simulink model "DWPT_simscape"  (R2026b)
settings: Solver=ode23t  StopTime=0.07  FixedStep=Ts  MaxStep=1.0E-7
InitFcn:
  | f = 85000;
  | Fs = 100000000;       % 100
  | Ts = 1/Fs;          % 步长
  | 
  | 
  | fprintf('周期/Ts = %.10f (应=100)\n', (1/f)/Ts);
  | 
  | 
  | LP1 = 437.3e-6;
  | LP2 = 420.6e-6;
  | LS = 306e-6;
  | LT1 = 98e-6;
  | LT2 = 99.5e-6;
  | 
  | CP1 = 9.03e-9;
  | CP2 = 9.23e-9;
  | 
  | CT1 = 55e-9;
  | CT2 = 54e-9;
  | CS = 12.5e-9;
  | 
  | M1  = 94e-6;
  | M2  = 0e-6;
  | 
  | RP1 = 1.4;
  | RP2 = 1.4;
  | RS = 1.3;
  | 
  | RL = 30;
undefined symbols (not defined in the file): Lf, Lt, M, Mosfet_class, MutualInductance_class, UniversalBridge_class
libraries: fl_lib x30, nesl_utility x23, ee_lib x9, eeRmsMeasurement x7, eeGeneralControl x3, dspfdesign x1, elec_conv_HighZElecRef x1, spspowerguiLib x1
(part 1 of 2)
settings Model: Creator=yihao  LastModifiedBy=rithvik
settings DataIOCC: ReturnWorkspaceOutputs=off
settings DebuggingCC: SaveWithParameterizedLinksMsg=none
settings RTWCC: GPUComputeCapability=5.0
settings SimscapeCC: SimscapeNominalValues="[{\"value\":\"1\",\"unit\":\"A\"},{\"value\":\"1\",\"unit\":\"bar\"},{\"value\":\"1\",\"unit\":\"cm^2\"},{\"value\":\"1\",\"unit\":\"cm^3/s\"},{\"value\":\"1\",\"unit\":\"kJ/kg\"},{\"value\":\"1\",\"unit\":\"kW\"},{\"value\":\"1\",\"unit\":\"l\"},{\"value\":\"1\",\"unit\":\"N\"},{\"value\":\"1\",\"unit\":\"N*m\"},{\"value\":\"1\",\"unit\":\"V\"},{\"value\":\"0.001\",\"unit\":\"Wb\"}]"  SimscapeUseEnergyAccounting=off

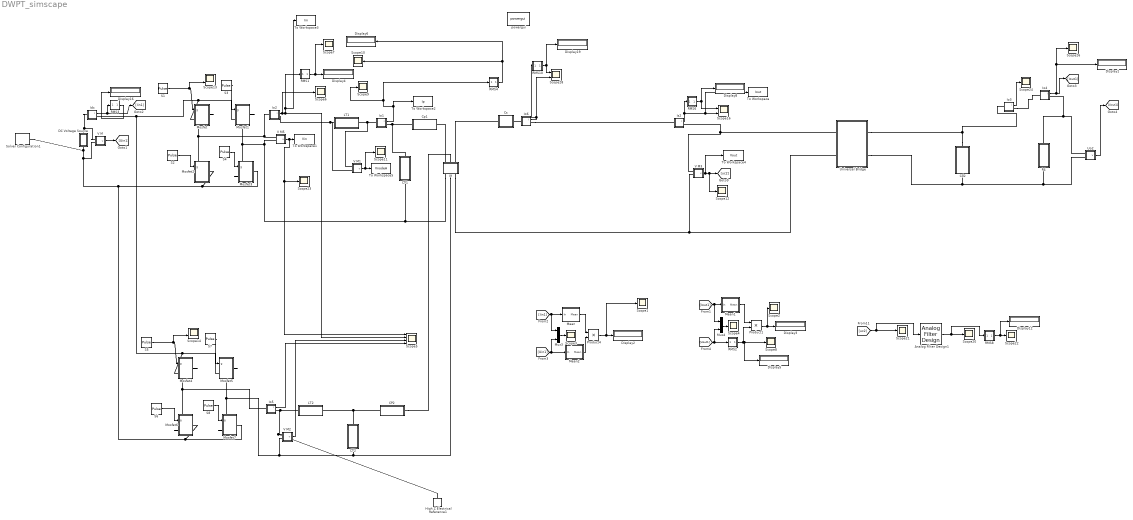
== system DWPT_simscape ==
  Analog Filter Design1 : dspfdesign/Analog Filter Design  method=Butterworth  filttype=Lowpass  N=8  Wlo=85000*2*pi  Whi=80  Rp=2  Rs=40
  CP2 : Subsystem
      settings: OpenFcn=elec.conv.unmask(gcb);
  CT1 : Subsystem
      settings: OpenFcn=elec.conv.unmask(gcb);
  CT2 : Subsystem
      settings: OpenFcn=elec.conv.unmask(gcb);
  Cd2 : Subsystem
      settings: OpenFcn=elec.conv.unmask(gcb);
  Cp1 : Subsystem
      settings: OpenFcn=elec.conv.unmask(gcb);
  Cs : Subsystem
      settings: OpenFcn=elec.conv.unmask(gcb);
  DC Voltage Source : Subsystem
      settings: OpenFcn=elec.conv.unmask(gcb);
  Display{1..6,8,12,16,19} (10 alike) : Display
  High Z Electrical Reference1 : elec_conv_HighZElecRef/High Z Electrical Reference  SystemSampleTime=-1  VariantActivationTime=update diagram  EmptyChoice=off  PassThrough=off  PassThroughVariantControl=(default)  EmptyChoiceVariantControl=(default)  AllowFlexibleInterface=on  Latency=0  AutoFrameSizeCalculation=off
  Idc : Subsystem
      settings: OpenFcn=elec.conv.unmask(gcb);
  Io1 : Subsystem
      settings: OpenFcn=elec.conv.unmask(gcb);
  Io2 : Subsystem
      settings: OpenFcn=elec.conv.unmask(gcb);
  Io3 : Subsystem
      settings: OpenFcn=elec.conv.unmask(gcb);
  Io4 : Subsystem
      settings: OpenFcn=elec.conv.unmask(gcb);
  Io5 : Subsystem
      settings: OpenFcn=elec.conv.unmask(gcb);
  Io6 : Subsystem
      settings: OpenFcn=elec.conv.unmask(gcb);
  Is2 : Subsystem
      settings: OpenFcn=elec.conv.unmask(gcb);
  LT1 : Subsystem
      settings: OpenFcn=elec.conv.unmask(gcb);
  LT2 : Subsystem
      settings: OpenFcn=elec.conv.unmask(gcb);
  M : Subsystem
      settings: AttributesFormatString=\n  OpenFcn=elec.conv.unmask(gcb);
  Mean : Subsystem
      settings: OpenFcn=elec.conv.unmask(gcb);
  Mean1 : Subsystem
      settings: OpenFcn=elec.conv.unmask(gcb);
  Mean2 : Subsystem
      settings: OpenFcn=elec.conv.unmask(gcb);
  Mosfet : Subsystem
      settings: OpenFcn=elec.conv.unmask(gcb);
  Mosfet1 : Subsystem
      settings: OpenFcn=elec.conv.unmask(gcb);
  Mosfet2 : Subsystem
      settings: OpenFcn=elec.conv.unmask(gcb);
  Mosfet3 : Subsystem
      settings: OpenFcn=elec.conv.unmask(gcb);
  Mosfet4 : Subsystem
      settings: OpenFcn=elec.conv.unmask(gcb);
  Mosfet5 : Subsystem
      settings: OpenFcn=elec.conv.unmask(gcb);
  Mosfet6 : Subsystem
      settings: OpenFcn=elec.conv.unmask(gcb);
  Mosfet7 : Subsystem
      settings: OpenFcn=elec.conv.unmask(gcb);
  Mux3 : Mux  Inputs=2
  Mux4 : Mux  Inputs=2
  Product1 : Product
  Product4 : Product
  R4 : Subsystem
      settings: OpenFcn=elec.conv.unmask(gcb);
  RMS1 : Subsystem
      settings: OpenFcn=elec.conv.unmask(gcb);
  RMS10 : Subsystem
      settings: OpenFcn=elec.conv.unmask(gcb);
  RMS2 : Subsystem
      settings: OpenFcn=elec.conv.unmask(gcb);
  RMS3 : Subsystem
      settings: OpenFcn=elec.conv.unmask(gcb);
  RMS4 : Subsystem
      settings: OpenFcn=elec.conv.unmask(gcb);
  RMS6 : Subsystem
      settings: OpenFcn=elec.conv.unmask(gcb);
  RMS8 : Subsystem
      settings: OpenFcn=elec.conv.unmask(gcb);
  S{1,4..5,8} (4 alike) : DiscretePulseGenerator  PulseType=Time based  Period=1/f  PulseWidth=49.5
  S{2..3,6..7} (4 alike) : DiscretePulseGenerator  PulseType=Time based  Period=1/f  PulseWidth=49.5  PhaseDelay=1/2/f
  Scope{1..4,6..12,20..24,26} (17 alike) : Scope
      Scope1 settings: ActiveDisplayYMinimum=-49.10464  ActiveDisplayYMaximum=441.94179  DataLoggingSaveFormat=Array
      Scope10 settings: ActiveDisplayYMinimum=-0.71464  ActiveDisplayYMaximum=6.43176  DataLoggingVariableName=ScopeData2  DataLoggingSaveFormat=Array
      Scope11 settings: ActiveDisplayYMinimum=-10.18584  ActiveDisplayYMaximum=11.18954  DataLoggingSaveFormat=Array
      Scope12 settings: ActiveDisplayYMinimum=-124.85082  ActiveDisplayYMaximum=124.97825  DataLoggingVariableName=ScopeData4  DataLoggingSaveFormat=Array
      Scope2 settings: ActiveDisplayYMinimum=-3.3359920538155139  ActiveDisplayYMaximum=30.023928484339635  DataLoggingVariableName=ScopeData12  DataLoggingSaveFormat=Array
      Scope20 settings: ActiveDisplayYMinimum=-998.97593  ActiveDisplayYMaximum=1003.83836  DataLoggingVariableName=ScopeData13  DataLoggingSaveFormat=Array
      Scope21 settings: ActiveDisplayYMinimum=-1098.42082  ActiveDisplayYMaximum=1097.9597  DataLoggingVariableName=ScopeData14  DataLoggingSaveFormat=Array
      Scope22 settings: ActiveDisplayYMinimum=-0.08617  ActiveDisplayYMaximum=0.77556  DataLoggingVariableName=ScopeData15  DataLoggingSaveFormat=Array
      Scope23 settings: ActiveDisplayYMinimum=-126.90541  ActiveDisplayYMaximum=126.90651  DataLoggingVariableName=ScopeData16  DataLoggingSaveFormat=Array
      Scope24 settings: ActiveDisplayYMinimum=-0.06956  ActiveDisplayYMaximum=0.62607  DataLoggingSaveFormat=Array
      Scope26 settings: ActiveDisplayYMinimum=-0.31456  ActiveDisplayYMaximum=2.83101  DataLoggingVariableName=ScopeData2  DataLoggingSaveFormat=Array
      Scope3 settings: ActiveDisplayYMinimum=-3742.24205  ActiveDisplayYMaximum=32139.40337  DataLoggingVariableName=ScopeData23  DataLoggingSaveFormat=Array
      Scope4 settings: ActiveDisplayYMinimum=-3.3830504056400548  ActiveDisplayYMaximum=30.4474536507605  DataLoggingVariableName=ScopeData27  DataLoggingSaveFormat=Array
      Scope6 settings: ActiveDisplayYMinimum=-10.18584  ActiveDisplayYMaximum=11.18954  DataLoggingVariableName=ScopeData29  DataLoggingSaveFormat=Array
      Scope7 settings: ActiveDisplayYMinimum=41.35748  ActiveDisplayYMaximum=44.91904  DataLoggingVariableName=ScopeData30  DataLoggingSaveFormat=Array
      Scope8 settings: ActiveDisplayYMinimum=-10.89533  ActiveDisplayYMaximum=134.54393  DataLoggingVariableName=ScopeData31  DataLoggingSaveFormat=Array
      Scope9 settings: ActiveDisplayYMinimum=-11.00674  ActiveDisplayYMaximum=11.77758  DataLoggingSaveFormat=Array
  Scope{13..14,16,28} (4 alike) : Scope  NumInputPorts=2
      Scope13 settings: ActiveDisplayYMinimum=-12.75848  ActiveDisplayYMaximum=112.74941  DataLoggingVariableName=ScopeData5  DataLoggingSaveFormat=Array
      Scope14 settings: ActiveDisplayYMinimum=-12.75848  ActiveDisplayYMaximum=112.74941  DataLoggingVariableName=ScopeData3  DataLoggingSaveFormat=Array
      Scope16 settings: ActiveDisplayYMinimum=-5.8521517419594016  ActiveDisplayYMaximum=5.8917781570828591  DataLoggingVariableName=ScopeData8  DataLoggingSaveFormat=Array
      Scope28 settings: ActiveDisplayYMinimum=-4.84326  ActiveDisplayYMaximum=4.41106  DataLoggingVariableName=ScopeData21  DataLoggingSaveFormat=Array
  Scope5 : Scope  NumInputPorts=4
      settings: ActiveDisplayYMinimum=-71.017946366553787  ActiveDisplayYMaximum=71.042097514829976  DataLoggingVariableName=ScopeData28  DataLoggingSaveFormat=Array
  Solver Configuration1 : nesl_utility/Solver Configuration  PhysicalDomain=network_engine_domain  SubClassName=solver  LeftPortType=input  RightPortType=generic  Tones=[]  Harmonics=[]  SimulateNoise=off  Profile=off  UseLocalSampling=off  EnableSwitchedLinearOptims=on  FrequencyDomain=off  UseCCode=off  RelTol=0.001  AbsTol=0.001  MinStep=1e-09  ToWorkspace=off  RevertToSquareIcSolve=off  NumHomotopyIterations=100  PhasorMode=off  PhasorModeNumHarmonics=1  ConsistencySolver=NEWTON_XTOL_AFTER_FTOL  CanonicalOrdering=CANONICAL  OptimizeIntermediates=OPTIMIZED  MulticoreSolverChoice=BACKWARD_EULER  IndexReductionMethod=DerivativeReplacement  DoDC=off  ResidualTolerance=1e-09  ConsistencyTolSource=GLOBAL  ConsistencyAbsTol=0.001  ConsistencyRelTol=0.001  ConsistencyTolFactor=0.001  UseLocalSolver=off  LocalSolverChoice=NE_BACKWARD_EULER_ADVANCER  ResolveIndetEquations=on  FunctionEvalNumThread=1  LocalSolverSampleTime=0.001  DoFixedCost=off  MaxNonlinIter=3  MaxModeIter=2  ComputeImpulses=off  ImpulseIterations=2  LinearAlgebra=auto  LinearAlgebraNumThread=0  EquationFormulation=NE_TIME_EF  DelaysMemoryBudget=1024  AutomaticFiltering=on  FilteringTimeConstant=0.001  PartitionStorageMethod=AS_NEEDED  PartitionMemoryBudget=1024  PartitionMethod=BALANCED  MultibodyUseLocalSolver=off  MultibodyLocalSolverChoice=ODE1  MultibodyLocalSolverSampleTime=0.001
  To Workspace : ToWorkspace  VariableName=Iout  SaveFormat=Structure With Time  SampleTime=-1
  To Workspace1 : ToWorkspace  VariableName=Vin  SaveFormat=Structure With Time  SampleTime=-1
  To Workspace2 : ToWorkspace  VariableName=Ip  SaveFormat=Structure With Time  SampleTime=-1
  To Workspace3 : ToWorkspace  VariableName=Iin  SaveFormat=Structure With Time  SampleTime=-1
  To Workspace4 : ToWorkspace  VariableName=Vout  SaveFormat=Structure With Time  SampleTime=-1
  To Workspace5 : ToWorkspace  VariableName=VnodeA  SaveFormat=Structure With Time  SampleTime=-1
  Universal Bridge : Subsystem
      settings: OpenFcn=elec.conv.unmask(gcb);
  Uo2 : Subsystem
      settings: OpenFcn=elec.conv.unmask(gcb);
  V M : Subsystem
      settings: OpenFcn=elec.conv.unmask(gcb);
  V M1 : Subsystem
      settings: OpenFcn=elec.conv.unmask(gcb);
  V M2 : Subsystem
      settings: OpenFcn=elec.conv.unmask(gcb);
  V M3 : Subsystem
      settings: OpenFcn=elec.conv.unmask(gcb);
  V M5 : Subsystem
      settings: OpenFcn=elec.conv.unmask(gcb);
  powergui : spspowerguiLib/powergui  Priority=1  SimulationMode=Discrete  SampleTime=1e-7  frequency=60  Iterations=50  frequencyindice=0  Pbase=100e6  ErrMax=1e-4  UnitsV=kV  UnitsW=MW  buscounter=0  FunctionMessages=off  echomessages=off  EnableUseOfTLC=off  CurrentSourceSwitches=off  DisableSnubberDevices=off  DisableRonSwitches=off  DisableVfSwitches=off  DisplayEquations=off  AutomaticDiscreteSolvers=off  SolverType=Tustin/Backward Euler (TBE)  Interpol=off  ExternalGateDelay=off  methode=off  Ts=100  x0status=blocks  SPID=on  SwTol=0  HookPort=off  NonlinearTolerance=1e-4  nMaxIteration=100  ContinueOnMaxIteration=off  RestoreLinks=warning  ResistiveCurrentMeasurement=off  Frange=[0:2:500]  Ylog=off  Xlog=on  ShowGrid=off  save=off  variable=ZData  structure=Is2  ZoomFFT=off  StartTime=0.1  cycles=5  DisplayStyle=1  fundamental=85000  FreqAxis=off  MaxFrequency=100000  frequencyindicesteady=1  RmsSteady=1  display=off
  wires:
  Is2/1(i) -> To Workspace/1, Scope16/2, RMS6/1(In)
  Io6/1(i) -> Scope28/2, RMS10/1(In)
  [Uin1] -> Mean2/1(In), Mux3/2
  V M5/1(v) -> To Workspace1/1, Scope5/1, Scope23/1
  [Uout1] -> RMS2/1(In), Mux4/2
  RMS4/1(RMS) -> Display6/1, Scope10/1
  Mean/1(Mean) -> Product4/1
  Idc/1(i) -> RMS3/1(In), [Iin1]
  V M3/1(v) -> To Workspace4/1, Scope12/1, [uc2]
  Mean1/1(Mean) -> Product1/1
  Io2/1(i) -> Scope5/2, To Workspace3/1, RMS1/1(In), Scope6/1
  [Iin1] -> Mean/1(In), Mux3/1
  S2/1 -> Mosfet2/1(g)
  RMS2/1(RMS) -> Display5/1, Scope8/1, Product1/2
  Mux4/1 -> Scope4/1
  Mean2/1(Mean) -> Product4/2
  [uc2] -> Analog Filter Design1/1, Scope21/1
  Product1/1 -> Scope2/1, Display3/1
  S4/1 -> Mosfet3/1(g)
  V M/1(v) -> [Uin1]
  Mux3/1 -> Scope3/1
  [Iout1] -> Mean1/1(In), Mux4/1
  RMS8/1(RMS) -> Display12/1, Scope22/1
  RMS1/1(RMS) -> Display4/1, Scope7/1
  Analog Filter Design1/1 -> RMS8/1(In), Scope20/1
  S1/1 -> Scope13/2, Mosfet/1(g)
  RMS6/1(RMS) -> Scope16/1, Display8/1
  Product4/1 -> Scope1/1, Display2/1
  RMS10/1(RMS) -> Scope28/1, Display19/1
  S3/1 -> Mosfet1/1(g)
  Io1/1(i) -> To Workspace2/1, RMS4/1(In), Scope9/1
  RMS3/1(RMS) -> Display16/1
  V M1/1(v) -> Scope11/1, To Workspace5/1
  Uo2/1(v) -> [Uout1]
  Io4/1(i) -> Display1/1, Scope26/1, [Iout1]
  Io3/1(i) -> Scope24/1
  V M2/1(v) -> Scope5/3
  Io5/1(i) -> Scope5/4
  S8/1 -> Mosfet7/1(g)
  S5/1 -> Scope14/2, Mosfet4/1(g)
  S6/1 -> Mosfet6/1(g)
  S7/1 -> Mosfet5/1(g)
  connections:
  Mosfet6/RConn1 -- V M/LConn2 -- DC Voltage Source/LConn1 -- Solver Configuration1/RConn1 -- Mosfet3/RConn1 -- Mosfet2/RConn1 -- Mosfet7/RConn1
  V M5/LConn1 -- Mosfet/RConn1 -- Mosfet2/LConn1 -- Io2/LConn1
  Idc/LConn1 -- DC Voltage Source/RConn1 -- V M/LConn1
  V M3/LConn1 -- Universal Bridge/LConn1 -- Is2/RConn1
  Io6/RConn1 -- Is2/LConn1
  Mosfet5/LConn1 -- Idc/RConn1 -- Mosfet/LConn1 -- Mosfet1/LConn1 -- Mosfet4/LConn1
  Io6/LConn1 -- Cs/LConn1
  Mosfet1/RConn1 -- Mosfet3/LConn1 -- CT1/RConn1 -- M/RConn1 -- V M5/LConn2
  M/LConn3 -- Cs/RConn1
  LT1/RConn1 -- V M1/LConn2 -- Io2/RConn1
  Io1/RConn1 -- CT1/LConn1 -- Cp1/RConn1
  Io1/LConn1 -- V M1/LConn1 -- LT1/LConn1
  Universal Bridge/LConn2 -- M/RConn3 -- V M3/LConn2
  Uo2/LConn1 -- R4/LConn1 -- Io4/RConn1
  Io3/RConn1 -- Io4/LConn1
  R4/RConn1 -- Uo2/LConn2 -- Cd2/RConn1 -- Universal Bridge/RConn2
  Cd2/LConn1 -- Io3/LConn1 -- Universal Bridge/RConn1
  CT2/LConn1 -- CP2/RConn1 -- LT2/LConn1
  CP2/LConn1 -- M/LConn2
  M/LConn1 -- Cp1/LConn1
  V M2/LConn1 -- High Z Electrical Reference1/LConn1 -- Io5/RConn1 -- LT2/RConn1
  Mosfet6/LConn1 -- Io5/LConn1 -- Mosfet4/RConn1
  Mosfet7/LConn1 -- V M2/LConn2 -- M/RConn2 -- CT2/RConn1 -- Mosfet5/RConn1

== system DWPT_simscape/CP2 ==
  Capacitor : fl_lib/Electrical/Electrical Elements/Capacitor  c=CP2 F  r=1e-6 Ohm  g=0 1/Ohm  i_specify=off  i_priority=None  i=0 A  i_nominal_specify=off  i_nominal_value=1  i_nominal_unit=A  v_specify=off  v_priority=None  v=0 V  v_nominal_specify=off  v_nominal_value=1  v_nominal_unit=V  vc_specify=on  vc_priority=None  vc=0 V  vc_nominal_specify=off  vc_nominal_value=1  vc_nominal_unit=V
  + : PMIOPort  Side=Left
  - : PMIOPort  Port=2  Side=Right
  connections:
  Capacitor/RConn1 -- -/RConn1
  +/RConn1 -- Capacitor/LConn1

== system DWPT_simscape/CT1 ==
  Capacitor : fl_lib/Electrical/Electrical Elements/Capacitor  c=CT1 F  r=1e-6 Ohm  g=0 1/Ohm  i_specify=off  i_priority=None  i=0 A  i_nominal_specify=off  i_nominal_value=1  i_nominal_unit=A  v_specify=off  v_priority=None  v=0 V  v_nominal_specify=off  v_nominal_value=1  v_nominal_unit=V  vc_specify=on  vc_priority=None  vc=0 V  vc_nominal_specify=off  vc_nominal_value=1  vc_nominal_unit=V
  + : PMIOPort  Side=Left
  - : PMIOPort  Port=2  Side=Right
  connections:
  Capacitor/RConn1 -- -/RConn1
  +/RConn1 -- Capacitor/LConn1

== system DWPT_simscape/CT2 ==
  Capacitor : fl_lib/Electrical/Electrical Elements/Capacitor  c=CT2 F  r=1e-6 Ohm  g=0 1/Ohm  i_specify=off  i_priority=None  i=0 A  i_nominal_specify=off  i_nominal_value=1  i_nominal_unit=A  v_specify=off  v_priority=None  v=0 V  v_nominal_specify=off  v_nominal_value=1  v_nominal_unit=V  vc_specify=on  vc_priority=None  vc=0 V  vc_nominal_specify=off  vc_nominal_value=1  vc_nominal_unit=V
  + : PMIOPort  Side=Left
  - : PMIOPort  Port=2  Side=Right
  connections:
  Capacitor/RConn1 -- -/RConn1
  +/RConn1 -- Capacitor/LConn1

== system DWPT_simscape/Cd2 ==
  Capacitor : fl_lib/Electrical/Electrical Elements/Capacitor  c=0.00047 F  r=1e-6 Ohm  g=0 1/Ohm  i_specify=off  i_priority=None  i=0 A  i_nominal_specify=off  i_nominal_value=1  i_nominal_unit=A  v_specify=off  v_priority=None  v=0 V  v_nominal_specify=off  v_nominal_value=1  v_nominal_unit=V  vc_specify=on  vc_priority=None  vc=0 V  vc_nominal_specify=off  vc_nominal_value=1  vc_nominal_unit=V
  + : PMIOPort  Side=Left
  - : PMIOPort  Port=2  Side=Right
  connections:
  Capacitor/RConn1 -- -/RConn1
  +/RConn1 -- Capacitor/LConn1

== system DWPT_simscape/Cp1 ==
  Capacitor : fl_lib/Electrical/Electrical Elements/Capacitor  c=CP1 F  r=1e-6 Ohm  g=0 1/Ohm  i_specify=off  i_priority=None  i=0 A  i_nominal_specify=off  i_nominal_value=1  i_nominal_unit=A  v_specify=off  v_priority=None  v=0 V  v_nominal_specify=off  v_nominal_value=1  v_nominal_unit=V  vc_specify=on  vc_priority=None  vc=0 V  vc_nominal_specify=off  vc_nominal_value=1  vc_nominal_unit=V
  + : PMIOPort  Side=Left
  - : PMIOPort  Port=2  Side=Right
  connections:
  Capacitor/RConn1 -- -/RConn1
  +/RConn1 -- Capacitor/LConn1

== system DWPT_simscape/Cs ==
  Capacitor : fl_lib/Electrical/Electrical Elements/Capacitor  c=CS F  r=1e-6 Ohm  g=0 1/Ohm  i_specify=off  i_priority=None  i=0 A  i_nominal_specify=off  i_nominal_value=1  i_nominal_unit=A  v_specify=off  v_priority=None  v=0 V  v_nominal_specify=off  v_nominal_value=1  v_nominal_unit=V  vc_specify=on  vc_priority=None  vc=0 V  vc_nominal_specify=off  vc_nominal_value=1  vc_nominal_unit=V
  + : PMIOPort  Side=Left
  - : PMIOPort  Port=2  Side=Right
  connections:
  Capacitor/RConn1 -- -/RConn1
  +/RConn1 -- Capacitor/LConn1

== system DWPT_simscape/DC Voltage Source ==
  DC Voltage Source : fl_lib/Electrical/Electrical Sources/DC Voltage Source  v0=50 V
  - : PMIOPort  Side=Left
  + : PMIOPort  Port=2  Side=Right
  connections:
  DC Voltage Source/RConn1 -- -/RConn1
  DC Voltage Source/LConn1 -- +/RConn1

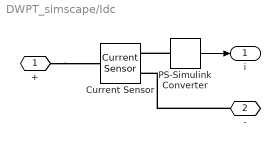
== system DWPT_simscape/Idc ==
  Current Sensor : fl_lib/Electrical/Electrical Sensors/Current Sensor
  PS-Simulink Converter : nesl_utility/PS-Simulink Converter  PhysicalDomain=network_engine_domain  SubClassName=ps_output  LeftPortType=input  RightPortType=output  PseudoPeriodic=off  Frequencies=[]  VectorFormat=1-D array  Unit=A  AffineConversion=off
  + : PMIOPort  Side=Left
  - : PMIOPort  Port=2  Side=Right
  i : Outport  VectorParamsAs1DForOutWhenUnconnected=off
  wires:
  PS-Simulink Converter/1 -> i/1
  connections:
  +/RConn1 -- Current Sensor/LConn1
  -/RConn1 -- Current Sensor/RConn2
  PS-Simulink Converter/LConn1 -- Current Sensor/RConn1

== system DWPT_simscape/Io1 ==
  Current Sensor : fl_lib/Electrical/Electrical Sensors/Current Sensor
  PS-Simulink Converter : nesl_utility/PS-Simulink Converter  PhysicalDomain=network_engine_domain  SubClassName=ps_output  LeftPortType=input  RightPortType=output  PseudoPeriodic=off  Frequencies=[]  VectorFormat=1-D array  Unit=A  AffineConversion=off
  + : PMIOPort  Side=Left
  - : PMIOPort  Port=2  Side=Right
  i : Outport  VectorParamsAs1DForOutWhenUnconnected=off
  wires:
  PS-Simulink Converter/1 -> i/1
  connections:
  +/RConn1 -- Current Sensor/LConn1
  -/RConn1 -- Current Sensor/RConn2
  PS-Simulink Converter/LConn1 -- Current Sensor/RConn1

== system DWPT_simscape/Io2 ==
  Current Sensor : fl_lib/Electrical/Electrical Sensors/Current Sensor
  PS-Simulink Converter : nesl_utility/PS-Simulink Converter  PhysicalDomain=network_engine_domain  SubClassName=ps_output  LeftPortType=input  RightPortType=output  PseudoPeriodic=off  Frequencies=[]  VectorFormat=1-D array  Unit=A  AffineConversion=off
  + : PMIOPort  Side=Left
  - : PMIOPort  Port=2  Side=Right
  i : Outport  VectorParamsAs1DForOutWhenUnconnected=off
  wires:
  PS-Simulink Converter/1 -> i/1
  connections:
  +/RConn1 -- Current Sensor/LConn1
  -/RConn1 -- Current Sensor/RConn2
  PS-Simulink Converter/LConn1 -- Current Sensor/RConn1

== system DWPT_simscape/Io3 ==
  Current Sensor : fl_lib/Electrical/Electrical Sensors/Current Sensor
  PS-Simulink Converter : nesl_utility/PS-Simulink Converter  PhysicalDomain=network_engine_domain  SubClassName=ps_output  LeftPortType=input  RightPortType=output  PseudoPeriodic=off  Frequencies=[]  VectorFormat=1-D array  Unit=A  AffineConversion=off
  + : PMIOPort  Side=Left
  - : PMIOPort  Port=2  Side=Right
  i : Outport  VectorParamsAs1DForOutWhenUnconnected=off
  wires:
  PS-Simulink Converter/1 -> i/1
  connections:
  +/RConn1 -- Current Sensor/LConn1
  -/RConn1 -- Current Sensor/RConn2
  PS-Simulink Converter/LConn1 -- Current Sensor/RConn1

== system DWPT_simscape/Io4 ==
  Current Sensor : fl_lib/Electrical/Electrical Sensors/Current Sensor
  PS-Simulink Converter : nesl_utility/PS-Simulink Converter  PhysicalDomain=network_engine_domain  SubClassName=ps_output  LeftPortType=input  RightPortType=output  PseudoPeriodic=off  Frequencies=[]  VectorFormat=1-D array  Unit=A  AffineConversion=off
  + : PMIOPort  Side=Left
  - : PMIOPort  Port=2  Side=Right
  i : Outport  VectorParamsAs1DForOutWhenUnconnected=off
  wires:
  PS-Simulink Converter/1 -> i/1
  connections:
  +/RConn1 -- Current Sensor/LConn1
  -/RConn1 -- Current Sensor/RConn2
  PS-Simulink Converter/LConn1 -- Current Sensor/RConn1

== system DWPT_simscape/Io5 ==
  Current Sensor : fl_lib/Electrical/Electrical Sensors/Current Sensor
  PS-Simulink Converter : nesl_utility/PS-Simulink Converter  PhysicalDomain=network_engine_domain  SubClassName=ps_output  LeftPortType=input  RightPortType=output  PseudoPeriodic=off  Frequencies=[]  VectorFormat=1-D array  Unit=A  AffineConversion=off
  + : PMIOPort  Side=Left
  - : PMIOPort  Port=2  Side=Right
  i : Outport  VectorParamsAs1DForOutWhenUnconnected=off
  wires:
  PS-Simulink Converter/1 -> i/1
  connections:
  +/RConn1 -- Current Sensor/LConn1
  -/RConn1 -- Current Sensor/RConn2
  PS-Simulink Converter/LConn1 -- Current Sensor/RConn1

== system DWPT_simscape/Io6 ==
  Current Sensor : fl_lib/Electrical/Electrical Sensors/Current Sensor
  PS-Simulink Converter : nesl_utility/PS-Simulink Converter  PhysicalDomain=network_engine_domain  SubClassName=ps_output  LeftPortType=input  RightPortType=output  PseudoPeriodic=off  Frequencies=[]  VectorFormat=1-D array  Unit=A  AffineConversion=off
  + : PMIOPort  Side=Left
  - : PMIOPort  Port=2  Side=Right
  i : Outport  VectorParamsAs1DForOutWhenUnconnected=off
  wires:
  PS-Simulink Converter/1 -> i/1
  connections:
  +/RConn1 -- Current Sensor/LConn1
  -/RConn1 -- Current Sensor/RConn2
  PS-Simulink Converter/LConn1 -- Current Sensor/RConn1

== system DWPT_simscape/Is2 ==
  Current Sensor : fl_lib/Electrical/Electrical Sensors/Current Sensor
  PS-Simulink Converter : nesl_utility/PS-Simulink Converter  PhysicalDomain=network_engine_domain  SubClassName=ps_output  LeftPortType=input  RightPortType=output  PseudoPeriodic=off  Frequencies=[]  VectorFormat=1-D array  Unit=A  AffineConversion=off
  + : PMIOPort  Side=Left
  - : PMIOPort  Port=2  Side=Right
  i : Outport  VectorParamsAs1DForOutWhenUnconnected=off
  wires:
  PS-Simulink Converter/1 -> i/1
  connections:
  +/RConn1 -- Current Sensor/LConn1
  -/RConn1 -- Current Sensor/RConn2
  PS-Simulink Converter/LConn1 -- Current Sensor/RConn1

== system DWPT_simscape/LT1 ==
  Inductor : fl_lib/Electrical/Electrical Elements/Inductor  l=LT1 H  r=0 Ohm  g=1e-9 1/Ohm  i_specify=off  i_priority=None  i=0 A  i_nominal_specify=off  i_nominal_value=1  i_nominal_unit=A  v_specify=off  v_priority=None  v=0 V  v_nominal_specify=off  v_nominal_value=1  v_nominal_unit=V  i_L_specify=on  i_L_priority=None  i_L=0 A  i_L_nominal_specify=off  i_L_nominal_value=1  i_L_nominal_unit=A
  Resistor : fl_lib/Electrical/Electrical Elements/Resistor  R=0.1 Ohm  i_specify=off  i_priority=None  i=0 A  i_nominal_specify=off  i_nominal_value=1  i_nominal_unit=A  v_specify=off  v_priority=None  v=0 V  v_nominal_specify=off  v_nominal_value=1  v_nominal_unit=V
  + : PMIOPort  Side=Left
  - : PMIOPort  Port=2  Side=Right
  connections:
  Inductor/LConn1 -- Resistor/RConn1
  +/RConn1 -- Resistor/LConn1
  Inductor/RConn1 -- -/RConn1

== system DWPT_simscape/LT2 ==
  Inductor : fl_lib/Electrical/Electrical Elements/Inductor  l=LT2 H  r=0 Ohm  g=1e-9 1/Ohm  i_specify=off  i_priority=None  i=0 A  i_nominal_specify=off  i_nominal_value=1  i_nominal_unit=A  v_specify=off  v_priority=None  v=0 V  v_nominal_specify=off  v_nominal_value=1  v_nominal_unit=V  i_L_specify=on  i_L_priority=None  i_L=0 A  i_L_nominal_specify=off  i_L_nominal_value=1  i_L_nominal_unit=A
  Resistor : fl_lib/Electrical/Electrical Elements/Resistor  R=0.1 Ohm  i_specify=off  i_priority=None  i=0 A  i_nominal_specify=off  i_nominal_value=1  i_nominal_unit=A  v_specify=off  v_priority=None  v=0 V  v_nominal_specify=off  v_nominal_value=1  v_nominal_unit=V
  + : PMIOPort  Side=Left
  - : PMIOPort  Port=2  Side=Right
  connections:
  Inductor/LConn1 -- Resistor/RConn1
  +/RConn1 -- Resistor/LConn1
  Inductor/RConn1 -- -/RConn1

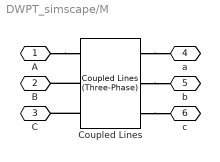
== system DWPT_simscape/M ==
  Coupled Lines : ee_lib/Passive/Lines/Coupled Lines (Three-Phase)  port_option=ee.enum.threePhasePort.expanded  prm=2  La="MutualInductance_class('Generalized mutual inductance','off',[0.06 Lf],[0.06 Lt],[1.1 0.0011],[0 M],3,[RP1  0 0; 0  RP2 0; 0 0 RS],[LP1 0 M1; 0 LP2 M2;M1 M2 LS]).objParamMappingDerived.NewDerivedParam.La H"  Lb="MutualInductance_class('Generalized mutual inductance','off',[0.06 Lf],[0.06 Lt],[1.1 0.0011],[0 M],3,[RP1  0 0; 0  RP2 0; 0 0 RS],[LP1 0 M1; 0 LP2 M2;M1 M2 LS]).objParamMappingDerived.NewDerivedParam.Lb H"  Lc="MutualInductance_class('Generalized mutual inductance','off',[0.06 Lf],[0.06 Lt],[1.1 0.0011],[0 M],3,[RP1  0 0; 0  RP2 0; 0 0 RS],[LP1 0 M1; 0 LP2 M2;M1 M2 LS]).objParamMappingDerived.NewDerivedParam.Lc H"  L=1e-3 H  Lmab="MutualInductance_class('Generalized mutual inductance','off',[0.06 Lf],[0.06 Lt],[1.1 0.0011],[0 M],3,[RP1  0 0; 0  RP2 0; 0 0 RS],[LP1 0 M1; 0 LP2 M2;M1 M2 LS]).objParamMappingDerived.NewDerivedParam.Lmab H"  Lmac="MutualInductance_class('Generalized mutual inductance','off',[0.06 Lf],[0.06 Lt],[1.1 0.0011],[0 M],3,[RP1  0 0; 0  RP2 0; 0 0 RS],[LP1 0 M1; 0 LP2 M2;M1 M2 LS]).objParamMappingDerived.NewDerivedParam.Lmac H"  Lmbc="MutualInductance_class('Generalized mutual inductance','off',[0.06 Lf],[0.06 Lt],[1.1 0.0011],[0 M],3,[RP1  0 0; 0  RP2 0; 0 0 RS],[LP1 0 M1; 0 LP2 M2;M1 M2 LS]).objParamMappingDerived.NewDerivedParam.Lmbc H"  Lm="MutualInductance_class('Generalized mutual inductance','off',[0.06 Lf],[0.06 Lt],[1.1 0.0011],[0 M],3,[RP1  0 0; 0  RP2 0; 0 0 RS],[LP1 0 M1; 0 LP2 M2;M1 M2 LS]).objParamMappingDerived.NewDerivedParam.Lm H"  Ra="MutualInductance_class('Generalized mutual inductance','off',[0.06 Lf],[0.06 Lt],[1.1 0.0011],[0 M],3,[RP1  0 0; 0  RP2 0; 0 0 RS],[LP1 0 M1; 0 LP2 M2;M1 M2 LS]).objParamMappingDerived.NewDerivedParam.Ra Ohm"  Rb="MutualInductance_class('Generalized mutual inductance','off',[0.06 Lf],[0.06 Lt],[1.1 0.0011],[0 M],3,[RP1  0 0; 0  RP2 0; 0 0 RS],[LP1 0 M1; 0 LP2 M2;M1 M2 LS]).objParamMappingDerived.NewDerivedParam.Rb Ohm"  Rc="MutualInductance_class('Generalized mutual inductance','off',[0.06 Lf],[0.06 Lt],[1.1 0.0011],[0 M],3,[RP1  0 0; 0  RP2 0; 0 0 RS],[LP1 0 M1; 0 LP2 M2;M1 M2 LS]).objParamMappingDerived.NewDerivedParam.Rc Ohm"  R=0.001 Ohm  Rmab=Rm Ohm  Rmac=Rm Ohm  Rmbc=Rm Ohm  Rm="MutualInductance_class('Generalized mutual inductance','off',[0.06 Lf],[0.06 Lt],[1.1 0.0011],[0 M],3,[RP1  0 0; 0  RP2 0; 0 0 RS],[LP1 0 M1; 0 LP2 M2;M1 M2 LS]).objParamMappingDerived.NewDerivedParam.Rm Ohm"  Ga=0 1/Ohm  Gb=0 1/Ohm  Gc=0 1/Ohm  G=1e-9 1/Ohm  I_L_specify=off  I_L_priority=High  I_L=[ 0 0 0 ] A  I_L_nominal_specify=off  I_L_nominal_value=1  I_L_nominal_unit=A  i_La_specify=off  i_La_priority=High  i_La=0 A  i_La_nominal_specify=off  i_La_nominal_value=1  i_La_nominal_unit=A  i_Lb_specify=off  i_Lb_priority=High  i_Lb=0 A  i_Lb_nominal_specify=off  i_Lb_nominal_value=1  i_Lb_nominal_unit=A  i_Lc_specify=off  i_Lc_priority=High  i_Lc=0 A  i_Lc_nominal_specify=off  i_Lc_nominal_value=1  i_Lc_nominal_unit=A
  A : PMIOPort  Side=Left
  B : PMIOPort  Port=2  Side=Left
  C : PMIOPort  Port=3  Side=Left
  a : PMIOPort  Port=4  Side=Right
  b : PMIOPort  Port=5  Side=Right
  c : PMIOPort  Port=6  Side=Right
  connections:
  Coupled Lines/LConn3 -- C/RConn1
  Coupled Lines/RConn3 -- c/RConn1
  Coupled Lines/RConn1 -- a/RConn1
  A/RConn1 -- Coupled Lines/LConn1
  Coupled Lines/RConn2 -- b/RConn1
  Coupled Lines/LConn2 -- B/RConn1

== system DWPT_simscape/Mean ==
  In : Inport
  Moving Average : eeGeneralControl/Moving Average  VariantControl=Variant1  LabelModeActiveChoice=Discrete  f=f/100  x0=0  BufferSize=8192  Ts=0
  Mean : Outport  VectorParamsAs1DForOutWhenUnconnected=off
  wires:
  Moving Average/1 -> Mean/1
  In/1 -> Moving Average/1

== system DWPT_simscape/Mean1 ==
  In : Inport
  Moving Average : eeGeneralControl/Moving Average  VariantControl=Variant1  LabelModeActiveChoice=Discrete  f=f  x0=0  BufferSize=8192  Ts=0
  Mean : Outport  VectorParamsAs1DForOutWhenUnconnected=off
  wires:
  Moving Average/1 -> Mean/1
  In/1 -> Moving Average/1

== system DWPT_simscape/Mean2 ==
  In : Inport
  Moving Average : eeGeneralControl/Moving Average  VariantControl=Variant1  LabelModeActiveChoice=Discrete  f=f/100  x0=0  BufferSize=8192  Ts=0
  Mean : Outport  VectorParamsAs1DForOutWhenUnconnected=off
  wires:
  Moving Average/1 -> Mean/1
  In/1 -> Moving Average/1

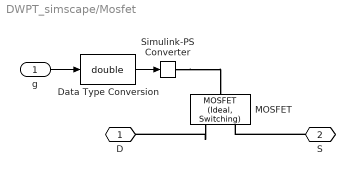
== system DWPT_simscape/Mosfet ==
  g : Inport
  Data Type Conversion : DataTypeConversion  OutDataTypeStr=double  SaturateOnIntegerOverflow=off  RndMeth=Floor
  MOSFET : ee_lib/Semiconductors & Converters/MOSFET (Ideal, Switching)  port_option=ee.enum.controlport.ps  Rds=Mosfet_class(0.01,100000,Inf,0.09,3.3).objParamMappingDerived.NewDerivedParam.Rds Ohm  Goff=Mosfet_class(0.01,100000,Inf,0.09,3.3).objParamMappingDerived.NewDerivedParam.Goff 1/Ohm  Vth=0.5 V  diode_param=2  diode_Vf=Mosfet_class(0.01,100000,Inf,0.09,3.3).objParamMappingDerived.NewDerivedParam.diode_Vf V  diode_Ron=Mosfet_class(0.01,100000,Inf,0.09,3.3).objParamMappingDerived.NewDerivedParam.diode_Ron Ohm  diode_Goff=Mosfet_class(0.01,100000,Inf,0.09,3.3).objParamMappingDerived.NewDerivedParam.diode_Goff 1/Ohm  diode_C=5e-8 F  diode_iRM=-235 A  diode_iF=300 A  diode_idot=-50 A/us  diode_trr_param=1  diode_trr_factor=3  diode_trr=15 us  diode_Qrr=1.5e+3 s*uA  ids_specify=off  ids_priority=None  ids=0 A  ids_nominal_specify=off  ids_nominal_value=1  ids_nominal_unit=A  vds_specify=off  vds_priority=None  vds=0 V  vds_nominal_specify=off  vds_nominal_value=1  vds_nominal_unit=V  vgs_specify=off  vgs_priority=None  vgs=0 V  vgs_nominal_specify=off  vgs_nominal_value=1  vgs_nominal_unit=V  thermal_loss_option=ee.enum.converters.thermalLossOption.constantvalues  Von_data=[0, 1.1, 1.3, 1.45, 1.75, 2.25, 2.7; 0, 1, 1.15, 1.35, 1.7, 2.35, 3] V  Tj=[298.15, 398.15] K  Iout_data=[0, 10, 50, 100, 200, 400, 600] A  tabulateWithVds=false  Eon_data=[0, .29, 1.43, 2.86, 5.71, 13.14, 22.86; 0, .57, 2.63, 5.14, 10.29, 20.57, 30.29] * 1e-3 J  Eoff_data=[0, .21, 1.07, 2.14, 4.29, 9.86, 17.14; 0, .43, 1.97, 3.86, 7.71, 15.43, 22.71] * 1e-3 J  Eon_data_3D=[zeros(2, 5, 3)] J  Eoff_data_3D=[zeros(2, 5, 3)] J  Tj_loss=[298.15, 448.15] K  Iout_data_loss=[0, 10, 20, 30, 40] A  Vds_loss=[0, 150, 300] V  Eon_scalar=22.86e-3 J  Eoff_scalar=17.14e-3 J  Voff=300 V  Iout_scalar=600 A  useCurrentFromPreviousCycle=true  currentMeasDelay=0 s  useVoltageFromPreviousCycle=true  voltageMeasDelay=0 s  diodeModelType=ee.enum.converters.diodeModelType.pwl  diodeTableType=ee.enum.diode.tableType.IfMat  diode_ReverseIVType=ee.enum.diode.diodeReverseIV.constant  diode_IfMat=[.07, .12, .19, 1.75, 4.24, 7.32, 11.2; .16, .3, .72, 2.14, 4.02, 6.35, 9.12] A  diode_VfMat=[.9, 1.15, 1.25, 1.5, 1.75, 2.17, 2.6, 2.85; .58, .68, .75, 1.1, 1.38, 1.77, 2.27, 2.7] V  diode_TjVec=[25, 125] degC  diode_VfVec=[.5, .7, .9, 1.3, 1.7, 2.1, 2.5] V  diode_IfVec=[.1, .2, .5, 1, 2, 4, 7, 10] A  diode_IrMat=[1e-06, 2e-06, 5e-06, 1e-05, 2.5e-05, 5e-05, .0001; 2e-06, 5e-06, 1e-05, 4e-05, 8e-05, .0002, .0005] A  diode_VrMat=[10, 100, 200, 250, 300, 325, 350; 10, 70, 160, 220, 270, 300, 320] V  diode_VrVec=[10, 20, 40, 50, 70, 80, 100] V  diode_IrVec=[1e-06, 2e-06, 5e-06, 1e-05, 2e-05, 5e-05, .0001] A  diode_Vr=-600 V  diode_Ls=150 nH  diode_Erec=0.03 J  diode_rec_loss_model=ee.enum.diode.reverseRecoveryModelTabulateUpTo3D.fixed  diode_ErecVal=0 J  diode_scaleWithIandV=true  diode_ErecMat=zeros(2, 3) J  diodeErecMat3D=zeros(2, 3, 2) J  diode_TjrecVec=[298.15, 398.15] K  diode_IfrecVec=[.1, 1, 10] A  diodeVrecVec=[0, 100] V  diode_IrecVal=10 A  diode_VrecVal=10 V  diode_tFilter=1 / 1000 / 100 s  separateThermalPortForDiode=false  thermal_network_parameterization=ee.enum.thermalNetworkTopology.external  Rth=[.03, .2] K/W  Rth_Cauer=[.03, .1, .2] K/W  Rth_Foster=[.03, .2] K/W  thermal_mass_parameterization=ee.enum.thermalNetwork.timeconstant  thermal_mass=[3, 25] J/K  thermal_mass_Cauer=[3, 10, 25] J/K  thermal_mass_Foster=[33, 50] J/K  thermal_time_constant=[.1, 5] s  thermal_time_constant_Cauer=[.1, 1, 5] s  thermal_time_constant_Foster=[1, 10] s  thermal_mass_initial_temperatures=[25, 25] degC  thermal_mass_initial_temperatures_Cauer=[25, 25, 25] degC  junction_thermal_mass=0.1 J/K  Tvec_initial_Foster=[25, 25, 25, 25] degC  RthDiode=[.03, .2] K/W  RthCauerDiode=[.03, .1, .2] K/W  RthFosterDiode=[.03, .2] K/W  thermalMassDiode=[3, 25] J/K  thermalMassCauerDiode=[3, 10, 25] J/K  thermalMassFosterDiode=[33, 50] J/K  thermalTauDiode=[.1, 5] s  thermalTauCauerDiode=[.1, 1, 5] s  thermalTauFosterDiode=[1, 10] s  thermalMassInitTempDiode=[25, 25] degC  thermalMassInitTempCauerDiode=[25, 25, 25] degC  junctionthermalMassDiode=0.1 J/K  TVecInitialFosterDiode=[25, 25] degC  no_thermal_network=ee.enum.enable.no  mosfet_junction_temperature_specify=off  mosfet_junction_temperature_priority=None  mosfet_junction_temperature=25 degC  mosfet_junction_temperature_nominal_specify=off  mosfet_junction_temperature_nominal_value=1  mosfet_junction_temperature_nominal_unit=degC  diode_junction_temperature_specify=off  diode_junction_temperature_priority=None  diode_junction_temperature=25 degC  diode_junction_temperature_nominal_specify=off  diode_junction_temperature_nominal_value=1  diode_junction_temperature_nominal_unit=degC  Qj_specify=off  Qj_priority=None  Qj=0 W  Qj_nominal_specify=off  Qj_nominal_value=1  Qj_nominal_unit=W  accumulatedSwitchingLosses_specify=off  accumulatedSwitchingLosses_priority=None  accumulatedSwitchingLosses=0 J
  Simulink-PS Converter : nesl_utility/Simulink-PS Converter  PhysicalDomain=network_engine_domain  SubClassName=ps_input  LeftPortType=input  RightPortType=output  PseudoPeriodic=off  Frequencies=[]  NoiseDistribution=none  NoiseParameters=[]  Unit=1  AffineConversion=off  FilteringAndDerivatives=provide  SimscapeFilterOrder=1  InputFilterTimeConstant=0.001  UdotUserProvided=0
  D : PMIOPort  Side=Left
  S : PMIOPort  Port=2  Side=Right
  wires:
  g/1 -> Data Type Conversion/1
  Data Type Conversion/1 -> Simulink-PS Converter/1
  connections:
  S/RConn1 -- MOSFET/RConn2
  Simulink-PS Converter/RConn1 -- MOSFET/LConn1
  MOSFET/RConn1 -- D/RConn1

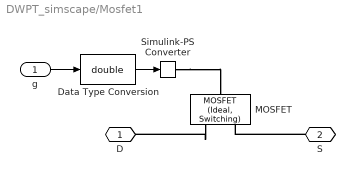
== system DWPT_simscape/Mosfet1 ==
  g : Inport
  Data Type Conversion : DataTypeConversion  OutDataTypeStr=double  SaturateOnIntegerOverflow=off  RndMeth=Floor
  MOSFET : ee_lib/Semiconductors & Converters/MOSFET (Ideal, Switching)  port_option=ee.enum.controlport.ps  Rds=Mosfet_class(0.01,100000,Inf,0.09,3.3).objParamMappingDerived.NewDerivedParam.Rds Ohm  Goff=Mosfet_class(0.01,100000,Inf,0.09,3.3).objParamMappingDerived.NewDerivedParam.Goff 1/Ohm  Vth=0.5 V  diode_param=2  diode_Vf=Mosfet_class(0.01,100000,Inf,0.09,3.3).objParamMappingDerived.NewDerivedParam.diode_Vf V  diode_Ron=Mosfet_class(0.01,100000,Inf,0.09,3.3).objParamMappingDerived.NewDerivedParam.diode_Ron Ohm  diode_Goff=Mosfet_class(0.01,100000,Inf,0.09,3.3).objParamMappingDerived.NewDerivedParam.diode_Goff 1/Ohm  diode_C=5e-8 F  diode_iRM=-235 A  diode_iF=300 A  diode_idot=-50 A/us  diode_trr_param=1  diode_trr_factor=3  diode_trr=15 us  diode_Qrr=1.5e+3 s*uA  ids_specify=off  ids_priority=None  ids=0 A  ids_nominal_specify=off  ids_nominal_value=1  ids_nominal_unit=A  vds_specify=off  vds_priority=None  vds=0 V  vds_nominal_specify=off  vds_nominal_value=1  vds_nominal_unit=V  vgs_specify=off  vgs_priority=None  vgs=0 V  vgs_nominal_specify=off  vgs_nominal_value=1  vgs_nominal_unit=V  thermal_loss_option=ee.enum.converters.thermalLossOption.constantvalues  Von_data=[0, 1.1, 1.3, 1.45, 1.75, 2.25, 2.7; 0, 1, 1.15, 1.35, 1.7, 2.35, 3] V  Tj=[298.15, 398.15] K  Iout_data=[0, 10, 50, 100, 200, 400, 600] A  tabulateWithVds=false  Eon_data=[0, .29, 1.43, 2.86, 5.71, 13.14, 22.86; 0, .57, 2.63, 5.14, 10.29, 20.57, 30.29] * 1e-3 J  Eoff_data=[0, .21, 1.07, 2.14, 4.29, 9.86, 17.14; 0, .43, 1.97, 3.86, 7.71, 15.43, 22.71] * 1e-3 J  Eon_data_3D=[zeros(2, 5, 3)] J  Eoff_data_3D=[zeros(2, 5, 3)] J  Tj_loss=[298.15, 448.15] K  Iout_data_loss=[0, 10, 20, 30, 40] A  Vds_loss=[0, 150, 300] V  Eon_scalar=22.86e-3 J  Eoff_scalar=17.14e-3 J  Voff=300 V  Iout_scalar=600 A  useCurrentFromPreviousCycle=true  currentMeasDelay=0 s  useVoltageFromPreviousCycle=true  voltageMeasDelay=0 s  diodeModelType=ee.enum.converters.diodeModelType.pwl  diodeTableType=ee.enum.diode.tableType.IfMat  diode_ReverseIVType=ee.enum.diode.diodeReverseIV.constant  diode_IfMat=[.07, .12, .19, 1.75, 4.24, 7.32, 11.2; .16, .3, .72, 2.14, 4.02, 6.35, 9.12] A  diode_VfMat=[.9, 1.15, 1.25, 1.5, 1.75, 2.17, 2.6, 2.85; .58, .68, .75, 1.1, 1.38, 1.77, 2.27, 2.7] V  diode_TjVec=[25, 125] degC  diode_VfVec=[.5, .7, .9, 1.3, 1.7, 2.1, 2.5] V  diode_IfVec=[.1, .2, .5, 1, 2, 4, 7, 10] A  diode_IrMat=[1e-06, 2e-06, 5e-06, 1e-05, 2.5e-05, 5e-05, .0001; 2e-06, 5e-06, 1e-05, 4e-05, 8e-05, .0002, .0005] A  diode_VrMat=[10, 100, 200, 250, 300, 325, 350; 10, 70, 160, 220, 270, 300, 320] V  diode_VrVec=[10, 20, 40, 50, 70, 80, 100] V  diode_IrVec=[1e-06, 2e-06, 5e-06, 1e-05, 2e-05, 5e-05, .0001] A  diode_Vr=-600 V  diode_Ls=150 nH  diode_Erec=0.03 J  diode_rec_loss_model=ee.enum.diode.reverseRecoveryModelTabulateUpTo3D.fixed  diode_ErecVal=0 J  diode_scaleWithIandV=true  diode_ErecMat=zeros(2, 3) J  diodeErecMat3D=zeros(2, 3, 2) J  diode_TjrecVec=[298.15, 398.15] K  diode_IfrecVec=[.1, 1, 10] A  diodeVrecVec=[0, 100] V  diode_IrecVal=10 A  diode_VrecVal=10 V  diode_tFilter=1 / 1000 / 100 s  separateThermalPortForDiode=false  thermal_network_parameterization=ee.enum.thermalNetworkTopology.external  Rth=[.03, .2] K/W  Rth_Cauer=[.03, .1, .2] K/W  Rth_Foster=[.03, .2] K/W  thermal_mass_parameterization=ee.enum.thermalNetwork.timeconstant  thermal_mass=[3, 25] J/K  thermal_mass_Cauer=[3, 10, 25] J/K  thermal_mass_Foster=[33, 50] J/K  thermal_time_constant=[.1, 5] s  thermal_time_constant_Cauer=[.1, 1, 5] s  thermal_time_constant_Foster=[1, 10] s  thermal_mass_initial_temperatures=[25, 25] degC  thermal_mass_initial_temperatures_Cauer=[25, 25, 25] degC  junction_thermal_mass=0.1 J/K  Tvec_initial_Foster=[25, 25, 25, 25] degC  RthDiode=[.03, .2] K/W  RthCauerDiode=[.03, .1, .2] K/W  RthFosterDiode=[.03, .2] K/W  thermalMassDiode=[3, 25] J/K  thermalMassCauerDiode=[3, 10, 25] J/K  thermalMassFosterDiode=[33, 50] J/K  thermalTauDiode=[.1, 5] s  thermalTauCauerDiode=[.1, 1, 5] s  thermalTauFosterDiode=[1, 10] s  thermalMassInitTempDiode=[25, 25] degC  thermalMassInitTempCauerDiode=[25, 25, 25] degC  junctionthermalMassDiode=0.1 J/K  TVecInitialFosterDiode=[25, 25] degC  no_thermal_network=ee.enum.enable.no  mosfet_junction_temperature_specify=off  mosfet_junction_temperature_priority=None  mosfet_junction_temperature=25 degC  mosfet_junction_temperature_nominal_specify=off  mosfet_junction_temperature_nominal_value=1  mosfet_junction_temperature_nominal_unit=degC  diode_junction_temperature_specify=off  diode_junction_temperature_priority=None  diode_junction_temperature=25 degC  diode_junction_temperature_nominal_specify=off  diode_junction_temperature_nominal_value=1  diode_junction_temperature_nominal_unit=degC  Qj_specify=off  Qj_priority=None  Qj=0 W  Qj_nominal_specify=off  Qj_nominal_value=1  Qj_nominal_unit=W  accumulatedSwitchingLosses_specify=off  accumulatedSwitchingLosses_priority=None  accumulatedSwitchingLosses=0 J
  Simulink-PS Converter : nesl_utility/Simulink-PS Converter  PhysicalDomain=network_engine_domain  SubClassName=ps_input  LeftPortType=input  RightPortType=output  PseudoPeriodic=off  Frequencies=[]  NoiseDistribution=none  NoiseParameters=[]  Unit=1  AffineConversion=off  FilteringAndDerivatives=provide  SimscapeFilterOrder=1  InputFilterTimeConstant=0.001  UdotUserProvided=0
  D : PMIOPort  Side=Left
  S : PMIOPort  Port=2  Side=Right
  wires:
  g/1 -> Data Type Conversion/1
  Data Type Conversion/1 -> Simulink-PS Converter/1
  connections:
  S/RConn1 -- MOSFET/RConn2
  Simulink-PS Converter/RConn1 -- MOSFET/LConn1
  MOSFET/RConn1 -- D/RConn1

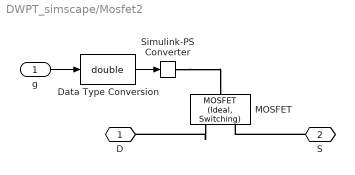
== system DWPT_simscape/Mosfet2 ==
  g : Inport
  Data Type Conversion : DataTypeConversion  OutDataTypeStr=double  SaturateOnIntegerOverflow=off  RndMeth=Floor
  MOSFET : ee_lib/Semiconductors & Converters/MOSFET (Ideal, Switching)  port_option=ee.enum.controlport.ps  Rds=Mosfet_class(0.01,100000,Inf,0.09,3.3).objParamMappingDerived.NewDerivedParam.Rds Ohm  Goff=Mosfet_class(0.01,100000,Inf,0.09,3.3).objParamMappingDerived.NewDerivedParam.Goff 1/Ohm  Vth=0.5 V  diode_param=2  diode_Vf=Mosfet_class(0.01,100000,Inf,0.09,3.3).objParamMappingDerived.NewDerivedParam.diode_Vf V  diode_Ron=Mosfet_class(0.01,100000,Inf,0.09,3.3).objParamMappingDerived.NewDerivedParam.diode_Ron Ohm  diode_Goff=Mosfet_class(0.01,100000,Inf,0.09,3.3).objParamMappingDerived.NewDerivedParam.diode_Goff 1/Ohm  diode_C=5e-8 F  diode_iRM=-235 A  diode_iF=300 A  diode_idot=-50 A/us  diode_trr_param=1  diode_trr_factor=3  diode_trr=15 us  diode_Qrr=1.5e+3 s*uA  ids_specify=off  ids_priority=None  ids=0 A  ids_nominal_specify=off  ids_nominal_value=1  ids_nominal_unit=A  vds_specify=off  vds_priority=None  vds=0 V  vds_nominal_specify=off  vds_nominal_value=1  vds_nominal_unit=V  vgs_specify=off  vgs_priority=None  vgs=0 V  vgs_nominal_specify=off  vgs_nominal_value=1  vgs_nominal_unit=V  thermal_loss_option=ee.enum.converters.thermalLossOption.constantvalues  Von_data=[0, 1.1, 1.3, 1.45, 1.75, 2.25, 2.7; 0, 1, 1.15, 1.35, 1.7, 2.35, 3] V  Tj=[298.15, 398.15] K  Iout_data=[0, 10, 50, 100, 200, 400, 600] A  tabulateWithVds=false  Eon_data=[0, .29, 1.43, 2.86, 5.71, 13.14, 22.86; 0, .57, 2.63, 5.14, 10.29, 20.57, 30.29] * 1e-3 J  Eoff_data=[0, .21, 1.07, 2.14, 4.29, 9.86, 17.14; 0, .43, 1.97, 3.86, 7.71, 15.43, 22.71] * 1e-3 J  Eon_data_3D=[zeros(2, 5, 3)] J  Eoff_data_3D=[zeros(2, 5, 3)] J  Tj_loss=[298.15, 448.15] K  Iout_data_loss=[0, 10, 20, 30, 40] A  Vds_loss=[0, 150, 300] V  Eon_scalar=22.86e-3 J  Eoff_scalar=17.14e-3 J  Voff=300 V  Iout_scalar=600 A  useCurrentFromPreviousCycle=true  currentMeasDelay=0 s  useVoltageFromPreviousCycle=true  voltageMeasDelay=0 s  diodeModelType=ee.enum.converters.diodeModelType.pwl  diodeTableType=ee.enum.diode.tableType.IfMat  diode_ReverseIVType=ee.enum.diode.diodeReverseIV.constant  diode_IfMat=[.07, .12, .19, 1.75, 4.24, 7.32, 11.2; .16, .3, .72, 2.14, 4.02, 6.35, 9.12] A  diode_VfMat=[.9, 1.15, 1.25, 1.5, 1.75, 2.17, 2.6, 2.85; .58, .68, .75, 1.1, 1.38, 1.77, 2.27, 2.7] V  diode_TjVec=[25, 125] degC  diode_VfVec=[.5, .7, .9, 1.3, 1.7, 2.1, 2.5] V  diode_IfVec=[.1, .2, .5, 1, 2, 4, 7, 10] A  diode_IrMat=[1e-06, 2e-06, 5e-06, 1e-05, 2.5e-05, 5e-05, .0001; 2e-06, 5e-06, 1e-05, 4e-05, 8e-05, .0002, .0005] A  diode_VrMat=[10, 100, 200, 250, 300, 325, 350; 10, 70, 160, 220, 270, 300, 320] V  diode_VrVec=[10, 20, 40, 50, 70, 80, 100] V  diode_IrVec=[1e-06, 2e-06, 5e-06, 1e-05, 2e-05, 5e-05, .0001] A  diode_Vr=-600 V  diode_Ls=150 nH  diode_Erec=0.03 J  diode_rec_loss_model=ee.enum.diode.reverseRecoveryModelTabulateUpTo3D.fixed  diode_ErecVal=0 J  diode_scaleWithIandV=true  diode_ErecMat=zeros(2, 3) J  diodeErecMat3D=zeros(2, 3, 2) J  diode_TjrecVec=[298.15, 398.15] K  diode_IfrecVec=[.1, 1, 10] A  diodeVrecVec=[0, 100] V  diode_IrecVal=10 A  diode_VrecVal=10 V  diode_tFilter=1 / 1000 / 100 s  separateThermalPortForDiode=false  thermal_network_parameterization=ee.enum.thermalNetworkTopology.external  Rth=[.03, .2] K/W  Rth_Cauer=[.03, .1, .2] K/W  Rth_Foster=[.03, .2] K/W  thermal_mass_parameterization=ee.enum.thermalNetwork.timeconstant  thermal_mass=[3, 25] J/K  thermal_mass_Cauer=[3, 10, 25] J/K  thermal_mass_Foster=[33, 50] J/K  thermal_time_constant=[.1, 5] s  thermal_time_constant_Cauer=[.1, 1, 5] s  thermal_time_constant_Foster=[1, 10] s  thermal_mass_initial_temperatures=[25, 25] degC  thermal_mass_initial_temperatures_Cauer=[25, 25, 25] degC  junction_thermal_mass=0.1 J/K  Tvec_initial_Foster=[25, 25, 25, 25] degC  RthDiode=[.03, .2] K/W  RthCauerDiode=[.03, .1, .2] K/W  RthFosterDiode=[.03, .2] K/W  thermalMassDiode=[3, 25] J/K  thermalMassCauerDiode=[3, 10, 25] J/K  thermalMassFosterDiode=[33, 50] J/K  thermalTauDiode=[.1, 5] s  thermalTauCauerDiode=[.1, 1, 5] s  thermalTauFosterDiode=[1, 10] s  thermalMassInitTempDiode=[25, 25] degC  thermalMassInitTempCauerDiode=[25, 25, 25] degC  junctionthermalMassDiode=0.1 J/K  TVecInitialFosterDiode=[25, 25] degC  no_thermal_network=ee.enum.enable.no  mosfet_junction_temperature_specify=off  mosfet_junction_temperature_priority=None  mosfet_junction_temperature=25 degC  mosfet_junction_temperature_nominal_specify=off  mosfet_junction_temperature_nominal_value=1  mosfet_junction_temperature_nominal_unit=degC  diode_junction_temperature_specify=off  diode_junction_temperature_priority=None  diode_junction_temperature=25 degC  diode_junction_temperature_nominal_specify=off  diode_junction_temperature_nominal_value=1  diode_junction_temperature_nominal_unit=degC  Qj_specify=off  Qj_priority=None  Qj=0 W  Qj_nominal_specify=off  Qj_nominal_value=1  Qj_nominal_unit=W  accumulatedSwitchingLosses_specify=off  accumulatedSwitchingLosses_priority=None  accumulatedSwitchingLosses=0 J
  Simulink-PS Converter : nesl_utility/Simulink-PS Converter  PhysicalDomain=network_engine_domain  SubClassName=ps_input  LeftPortType=input  RightPortType=output  PseudoPeriodic=off  Frequencies=[]  NoiseDistribution=none  NoiseParameters=[]  Unit=1  AffineConversion=off  FilteringAndDerivatives=provide  SimscapeFilterOrder=1  InputFilterTimeConstant=0.001  UdotUserProvided=0
  D : PMIOPort  Side=Left
  S : PMIOPort  Port=2  Side=Right
  wires:
  g/1 -> Data Type Conversion/1
  Data Type Conversion/1 -> Simulink-PS Converter/1
  connections:
  S/RConn1 -- MOSFET/RConn2
  Simulink-PS Converter/RConn1 -- MOSFET/LConn1
  MOSFET/RConn1 -- D/RConn1
